simulink model "MPA_04_ensayos"  (R2026a)
settings: Solver=FixedStepAuto  StopTime=280  FixedStep=0.02
InitFcn:
  | if exist('cal_MPA04.mat', 'file')
  |     load('cal_MPA04.mat')
  | else
  |     a2 = 0;  a1 = 1;  a0 = 0;      % sin calibrar: y_deg muestra las cuentas
  |     warning('Sin cal_MPA04.mat: corran calibracion_sensor.m (manual, sección 6).')
  | end
libraries: instrumentseriallib x3
settings Model: Creator=Sergio  LastModifiedBy=sergio.castano

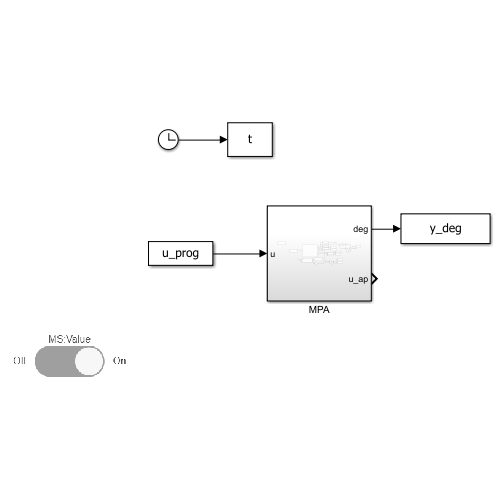
[thumbnail: Simulink's stored preview of the top-level diagram]
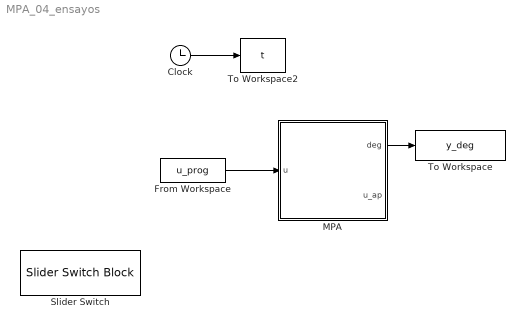
== system MPA_04_ensayos ==
  Clock : Clock
  From Workspace : FromWorkspace  VariableName=u_prog  SampleTime=0.02  Interpolate=off  OutputAfterFinalValue=Holding final value
  MPA : Subsystem
  Slider Switch : SliderSwitchBlock
  To Workspace : ToWorkspace  VariableName=y_deg  SampleTime=0.02
  To Workspace2 : ToWorkspace  VariableName=t  SampleTime=0.01
      settings: Save2DSignal=2-D array (concatenate along first dimension)
  wires:
  Clock/1 -> To Workspace2/1
  MPA/1(deg) -> To Workspace/1
  From Workspace/1 -> MPA/1(u)

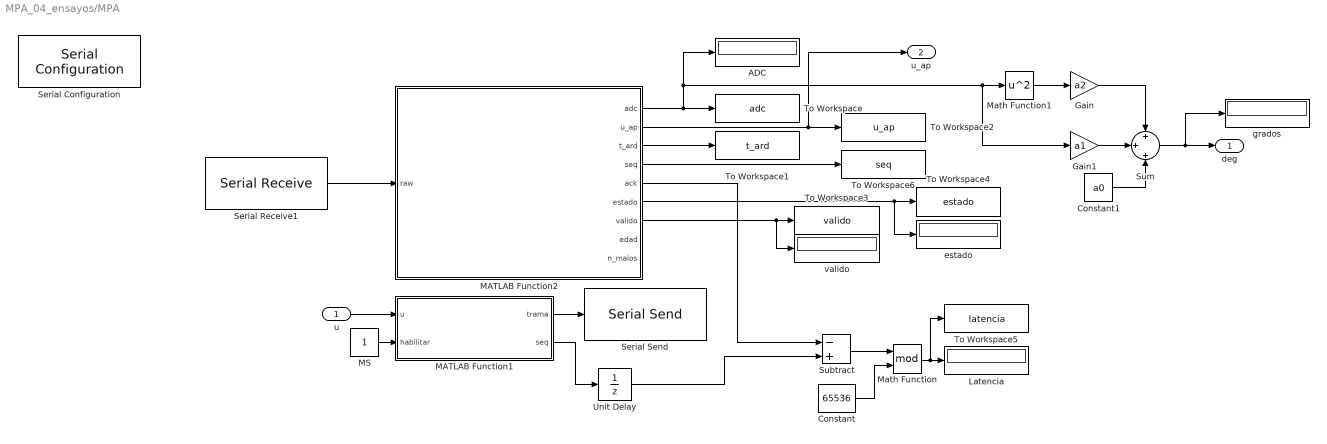
== system MPA_04_ensayos/MPA ==
  u : Inport
  ADC : Display
  Constant : Constant  Value=65536
  Constant1 : Constant  Value=a0
  Gain : Gain  Gain=a2
  Gain1 : Gain  Gain=a1
  Latencia : Display
  MATLAB Function1 : MATLAB Function  TreatAsAtomicUnit=on
  MATLAB Function2 : MATLAB Function  TreatAsAtomicUnit=on
  MS : Constant
  Math Function : Math  Operator=mod
  Math Function1 : Math  Operator=square
  Serial Configuration : instrumentseriallib/Serial Configuration  Priority=-200000  PortSel=COM26  Port=COM26  ComPort=COM26  BaudRate=115200  DataBits=8  Parity=none  StopBits=1  ByteOrder=little-endian  FlowControl=none  Timeout=10  SimulateUsing=Interpreted execution  BlockInModel=on  aMode=1
  Serial Receive1 : instrumentseriallib/Serial Receive  Priority=1  PortSel=COM26  Port=COM26  ComPort=COM26  ObjConstructor="\"serial('COM4');\""  DataType=uint8  SaveDataType=uint8  ToggleHeader=off  Header=[]  ToggleDataSize=on  DataSize=[22 1]  ToggleTerminator=off  Terminator=<none>  CustomTerminator=[]  InputFormat=Column major  EnableBlockingMode=on  ActionDataUnavailable=Output last received value  ActionWhenDataUnavailable=Output last received value  CustomValue=0  SampleTime=0.02  SimulateUsing=Interpreted execution  BlockInModel=on  aMode=1  LibraryInUse=instrumentlib
  Serial Send : instrumentseriallib/Serial Send  Priority=1  PortSel=COM26  Port=COM26  ComPort=COM26  Header=[]  Terminator=<none>  CustomTerminator=[]  EnableBlockingMode=on  SimulateUsing=Interpreted execution  BlockInModel=on  aMode=1
  Subtract : Sum  Inputs=-+
  Sum : Sum  Inputs=+|+|+
  To Workspace : ToWorkspace  VariableName=adc  SampleTime=0.02
  To Workspace1 : ToWorkspace  VariableName=t_ard  SampleTime=0.02
  To Workspace2 : ToWorkspace  VariableName=u_ap  SampleTime=0.02
  To Workspace3 : ToWorkspace  VariableName=valido  SampleTime=0.02
  To Workspace4 : ToWorkspace  VariableName=estado  SampleTime=0.02
  To Workspace5 : ToWorkspace  VariableName=latencia  SampleTime=0.02
  To Workspace6 : ToWorkspace  VariableName=seq  SampleTime=0.02
  Unit Delay : UnitDelay  SampleTime=-1
  estado : Display
  grados : Display
  valido : Display
  deg : Outport
  u_ap : Outport  Port=2
  wires:
  u/1 -> MATLAB Function1/1(u)
  MATLAB Function1/1(trama) -> Serial Send/1
  MS/1 -> MATLAB Function1/2(habilitar)
  MATLAB Function1/2(seq) -> Unit Delay/1
  MATLAB Function2/5(ack) -> Subtract/1
  Unit Delay/1 -> Subtract/2
  Subtract/1 -> Math Function/1
  Constant/1 -> Math Function/2
  Math Function/1 -> To Workspace5/1, Latencia/1
  MATLAB Function2/1(adc) -> ADC/1, Gain1/1, Math Function1/1, To Workspace/1
  MATLAB Function2/3(t_ard) -> To Workspace1/1
  MATLAB Function2/2(u_ap) -> u_ap/1, To Workspace2/1
  MATLAB Function2/7(valido) -> valido/1, To Workspace3/1
  MATLAB Function2/6(estado) -> estado/1, To Workspace4/1
  Serial Receive1/1 -> MATLAB Function2/1(raw)
  Math Function1/1 -> Gain/1
  Gain/1 -> Sum/1
  Gain1/1 -> Sum/2
  Constant1/1 -> Sum/3
  Sum/1 -> grados/1, deg/1
  MATLAB Function2/4(seq) -> To Workspace6/1

== matlab function MPA_04_ensayos/MPA/MATLAB Function1 ==
  data: u input; trama output; habilitar input; seq output
function [trama, seq] = packMPA(u, habilitar)
%#codegen
% packMPA  Arma el comando para el MPA (bloque MATLAB Function).
%
% Entradas: u          mando [%] (despues de la saturacion del modelo)
%           habilitar  1 = marcha permitida, 0 = PARO (motor detenido)
% Salidas:  trama      11x1 uint8 hacia el bloque Serial Send
%                      (Header vacio, Terminator <none>)
%           seq        numero de este comando (para medir la latencia con ack)
%
% Trama: 0xCC 0xDD | seq uint16 | u single | flags uint8 | crc16 (little-endian)
% El Arduino recorta u a [0,100] y tiene su propio tope de pulso; aqui
% tambien se recorta para que NaN o valores absurdos nunca salgan del PC.

persistent s
if isempty(s)
    s = 0;
end
s = mod(s + 1, 65536);                 % uint16 en MATLAB satura; aqui se envuelve

if ~isfinite(u)
    u = 0;
end
u = min(max(u, 0), 100);
fl = uint8(0);
if habilitar > 0.5
    fl = uint8(1);
end

carga = [typecast(uint16(s), 'uint8'), typecast(single(u), 'uint8'), fl];   % 7 bytes
trama = zeros(11, 1, 'uint8');
trama(1) = uint8(204);                 % 0xCC
trama(2) = uint8(221);                 % 0xDD
for k = 1:7
    trama(2+k) = carga(k);
end
c = crc16(carga);
trama(10) = uint8(mod(c, 256));
trama(11) = uint8(floor(c / 256));
seq = s;
end

% ---------------------------------------------------------------------
function c = crc16(d)
% CRC-16/CCITT-FALSE: polinomio 0x1021, inicial 0xFFFF (el mismo del Arduino)
r = uint16(65535);
for k = 1:numel(d)
    r = bitxor(r, bitshift(uint16(d(k)), 8));
    for b = 1:8
        if bitand(r, uint16(32768)) ~= 0
            r = bitxor(bitshift(r, 1), uint16(4129));
        else
            r = bitshift(r, 1);
        end
    end
end
c = double(r);
end

== matlab function MPA_04_ensayos/MPA/MATLAB Function2 ==
  data: raw input; adc output double; u_ap output double; t_ard output double; seq output; ack output; estado output; valido output; edad output; n_malos output
function [adc, u_ap, t_ard, seq, ack, estado, valido, edad, n_malos] = parseMPA(raw)
%#codegen
% parseMPA  Decodifica la telemetria del MPA (bloque MATLAB Function).
%
% Entrada:  raw  22x1 uint8, salida del bloque Serial Receive
%           (Header vacio, Terminator <none>, Data size [22 1], uint8,
%            modo bloqueante, Block sample time = Ts = 0.02).
% Salidas:  adc      promedio de cuentas de A0 (va a la calibracion)
%           u_ap     mando que el Arduino aplico de verdad [%]
%           t_ard    reloj del Arduino [s] (tiempo real del ensayo)
%           seq      numero del paquete leido
%           ack      ultimo comando que el Arduino acepto (para la latencia)
%           estado   1 = MARCHA, 0 = SEGURO (motor detenido)
%           valido   1 si hay paquete reciente; 0 si las salidas son el ultimo
%                    valor retenido (el lazo no debe confiar en esa medida)
%           edad     pasos seguidos sin paquete nuevo
%           n_malos  lecturas en que habia cabecera pero ningun paquete con
%                    CRC correcto (desde el inicio). Debe quedarse en 0 o casi.
%
% No supone que los 22 bytes leidos esten alineados con un paquete: guarda
% los ultimos 64 bytes y busca, de atras hacia adelante, el paquete mas
% reciente con cabecera 0xAA 0xBB y CRC-16 correcto. Asi se recupera solo
% de un arranque a mitad de paquete o de un byte perdido.

L  = 22;          % largo del paquete
NB = 64;          % memoria de bytes (cabe un paquete completo en cualquier desfase)
EDAD_MAX = 5;     % pasos sin paquete nuevo antes de declarar invalido (0.1 s)

persistent buf adc_m u_m t_m seq_m ack_m est_m nmal ed hay
if isempty(buf)
    buf  = zeros(NB, 1, 'uint8');
    adc_m = 0; u_m = 0; t_m = 0; seq_m = -1; ack_m = 0; est_m = 0;
    nmal = 0; ed = 0; hay = false;
end

% --- desplazar la memoria y agregar los bytes nuevos
r = uint8(raw(:));
for k = 1:NB-L
    buf(k) = buf(k+L);
end
for k = 1:L
    buf(NB-L+k) = r(k);
end

% --- buscar el paquete valido mas reciente
f = zeros(L, 1, 'uint8');
encontrado = false;
candidatos = 0;
for i = NB-L+1:-1:1
    if buf(i) == 170 && buf(i+1) == 187
        candidatos = candidatos + 1;
        for k = 1:L
            f(k) = buf(i+k-1);
        end
        if crc16(f(3:L-2)) == double(f(L-1)) + 256*double(f(L))
            encontrado = true;
            break
        end
    end
end
if candidatos > 0 && ~encontrado
    nmal = nmal + 1;
end

nuevo = false;
if encontrado
    sq = double(f(3)) + 256*double(f(4));                  % uint16, little-endian
    if sq ~= seq_m                      % paquete distinto al ya entregado
        nuevo = true;
        seq_m = sq;
        t_m   = (double(f(5)) + 256*double(f(6)) + 65536*double(f(7)) ...
                 + 16777216*double(f(8))) / 1000;           % uint32 [ms] -> s
        adc_m = bytesAFloat(f(9), f(10), f(11), f(12));
        u_m   = bytesAFloat(f(13), f(14), f(15), f(16));
        ack_m = double(f(17)) + 256*double(f(18));
        est_m = double(bitand(f(19), uint8(1)));
        hay   = true;
    end
end

if nuevo
    ed = 0;
else
    ed = ed + 1;
end

adc = adc_m;  u_ap = double(u_m);  t_ard = t_m;
seq = max(seq_m, 0);  ack = ack_m;  estado = est_m;
valido = double(hay && ed <= EDAD_MAX);
edad = ed;  n_malos = nmal;
end

% ---------------------------------------------------------------------
function x = bytesAFloat(b1, b2, b3, b4)
% 4 bytes little-endian -> single -> double (escalar fijo para el generador de codigo)
v = zeros(1, 4, 'uint8');
v(1) = b1;  v(2) = b2;  v(3) = b3;  v(4) = b4;
y = typecast(v, 'single');
x = double(y(1));
end

% ---------------------------------------------------------------------
function c = crc16(d)
% CRC-16/CCITT-FALSE: polinomio 0x1021, inicial 0xFFFF (el mismo del Arduino)
r = uint16(65535);
for k = 1:numel(d)
    r = bitxor(r, bitshift(uint16(d(k)), 8));
    for b = 1:8
        if bitand(r, uint16(32768)) ~= 0
            r = bitxor(bitshift(r, 1), uint16(4129));   % 0x1021; en uint16 los bits que salen se pierden
        else
            r = bitshift(r, 1);
        end
    end
end
c = double(r);
end
